simulink model "rlQuadrupedRobot"  (R2024b)
settings: Solver=ode23tb  StartTime=0.0  StopTime=10.0  RelTol=1e-3
values from neighbouring files (symbols this model uses):
  friction_force_max = mu_static * normal_force_max    [initializeRobotParameters.m]
  g = -9.81    [initializeRobotParameters.m]
  h_final = 0.75    [initializeRobotParameters.m]
  hip_eq_angle = 0    [initializeRobotParameters.m]
  init_ang_FL = d2r * quadrupedInverseKinematics(init_foot_disp_x,-init_body_height,l1,l2)    [initializeRobotParameters.m]
  init_ang_FR = init_ang_FL    [initializeRobotParameters.m]
  init_ang_RL = init_ang_FL    [initializeRobotParameters.m]
  init_ang_RR = init_ang_FL    [initializeRobotParameters.m]
  knee_eq_angle = 0    [initializeRobotParameters.m]
  l1 = 0.5517    [initializeRobotParameters.m]
  l2 = 0.5517    [initializeRobotParameters.m]
  L_back = 1.5    [initializeRobotParameters.m]
  M = 2    [initializeRobotParameters.m]
  m1 = 0.2    [initializeRobotParameters.m]
  m2 = 0.2    [initializeRobotParameters.m]
  normal_force_max = ((M+4*m1+4*m2)*abs(g))/4    [initializeRobotParameters.m]
  pitch_max = 10 * d2r    (= 0.174532925199)    [initializeRobotParameters.m]
  q_hip_max = -30 * d2r    (= -0.523598775598)    [initializeRobotParameters.m]
  q_hip_min = -120 * d2r    (= -2.09439510239)    [initializeRobotParameters.m]
  q_knee_max = 140 * d2r    (= 2.44346095279)    [initializeRobotParameters.m]
  q_knee_min = 60 * d2r    (= 1.0471975512)    [initializeRobotParameters.m]
  roll_max = 10 * d2r    (= 0.174532925199)    [initializeRobotParameters.m]
  Tf = 10    [initializeRobotParameters.m]
  Ts = 0.025    [initializeRobotParameters.m]
  u_max = 10    [initializeRobotParameters.m]
  vx_max = 2.5    [initializeRobotParameters.m]
  vy_max = 2.5    [initializeRobotParameters.m]
  vz_max = 2.5    [initializeRobotParameters.m]
  w_max = 2*pi*60/60    (= 6.28318530718)    [initializeRobotParameters.m]
  y_max = l1*cos(q_hip_max) + l2*cos(q_hip_max+q_knee_min)    [initializeRobotParameters.m]
  y_min = 0.5    [initializeRobotParameters.m]
  yaw_max = 20 * d2r    (= 0.349065850399)    [initializeRobotParameters.m]
  z_max = 0.5    [initializeRobotParameters.m]
undefined symbols (not defined in the file or in its folder): Extr_Data_LinkEndHole, Extr_Data_Mesh, ground, joint, X, Y, Z
libraries: sm_lib x113, nesl_utility x43, simulink x4, rllib x1
(part 1 of 5)
settings Model: Creator=The MathWorks, Inc.  LastModifiedBy=HP
settings SolverCC: AlgebraicLoopSolver=TrustRegion  MaxZcPerStep=1
settings OptimizationCC: ReuseModelBlockBuffer=off
settings DebuggingCC: UnconnectedInputMsg=warning  UnconnectedOutputMsg=warning  UnconnectedLineMsg=warning
settings ModelReferenceCC: EnableRefExpFcnMdlSchedulingChecks=on
settings SFSimCC: UsePrecompiledLibraries=Avoid  SimTargetLang=C++  GPUAcceleration=on  SimDLTargetLibrary=cudnn
settings RTWCC: GPUComputeCapability=3.5  DLArmComputeVersion=19.05
settings ExplorerConfigSet: InternalSimMechanicsExplorerSettings="<ExplorerConfiguration><canonicalview>default</canonicalview><AnimationSetting><BasePlaybackSpeed>1.0</BasePlaybackSpeed><PlaybackSpeedFactor>1.0</PlaybackSpeedFactor></AnimationSetting><TilePanel><TileInfo><Tiles Columns=\"1\" Count=\"1\" Rows=\"1\"><Column Weight=\"1\"/><Row Weight=\"1\"/><Tile Height=\"1\" Width=\"1\" X=\"0\" Y=\"0\"/></Tiles></TileInfo><SceneInfo><SceneViewer><BGColor><R>0.800000011920928955</R><G>0.800000011920928955</G><B>0.800000011920928955</B></BGColor><Camera><DoPerspective>off</DoPerspective><Position><X>43.366071430974273</X><Y>18.5858741674419576</Y><Z>23.6715179374704263</Z></Position><Center><X>3.63321843239613607</X><Y>-0.0564675288840452705</Y><Z>-0.89357222944397563</Z></Center><Up><X>-0.257452576685770707</X><Y>0.923486599880072756</Y><Z>-0.284412852381534909</Z></Up><ViewLimDist>1</ViewLimDist><YLim>2.82644414590933035</YLim><XLim>4.39998973134204618</XLim></Camera></SceneViewer></SceneInfo></TilePanel><MechEditorPanel><Cameras/><GfxPanelCameraMap/><VideoCreator><PlaybackSpeedRatio>1.0</PlaybackSpeedRatio><FrameRate>30</FrameRate><VideoFormat>Motion JPEG AVI</VideoFormat><FrameSize>auto</FrameSize></VideoCreator></MechEditorPanel></ExplorerConfiguration>"

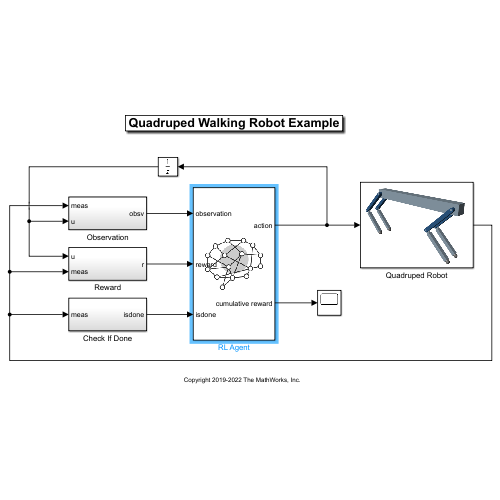
[thumbnail: Simulink's stored preview of the top-level diagram]
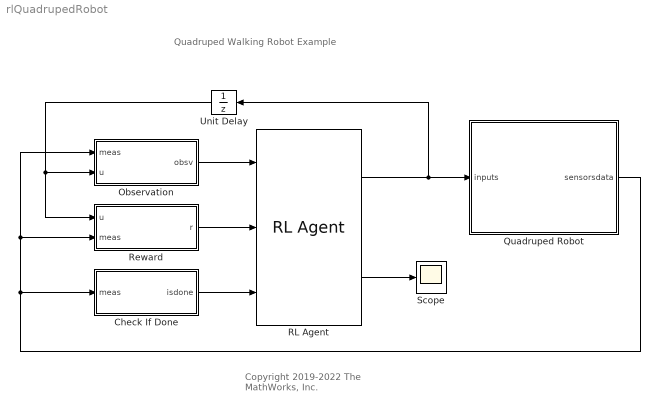
== system rlQuadrupedRobot ==
  note: Copyright 2019-2022 The MathWorks, Inc.
  note: Quadruped Walking Robot Example
  Check If Done : Subsystem
  Observation : Subsystem
  Quadruped Robot : Subsystem
      mask Display: image('$imagefile'); % Use "Edit Image" on toolstrip to change.
  RL Agent : rllib/RL Agent  Agent=agent1_Trained  ExternalActionAsInput=off  ProvideLastAction=off  ProvideCumRwd=on  TreatAsDirectFeedthrough=on  UseStrictObservationDataTypes=off
  Reward : Subsystem
  Scope : Scope
  Unit Delay : UnitDelay  SampleTime=-1  HasFrameUpgradeWarning=on
  wires:
  RL Agent/1 -> Quadruped Robot/1(inputs), Unit Delay/1
  Reward/1(r) -> RL Agent/2
  Unit Delay/1 -> Observation/2(u), Reward/1(u)
  RL Agent/2 -> Scope/1
  Quadruped Robot/1(sensorsdata) -> Observation/1(meas), Reward/2(meas), Check If Done/1(meas)
  Check If Done/1(isdone) -> RL Agent/3
  Observation/1(obsv) -> RL Agent/1

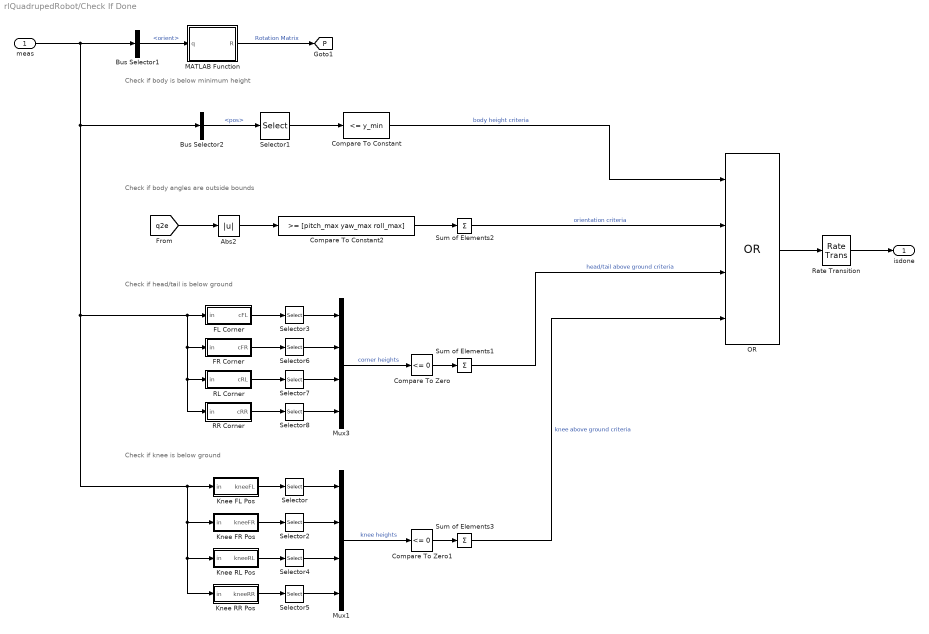
== system rlQuadrupedRobot/Check If Done ==
  note: Check if body is below minimum height
  note: Check if head/tail is below ground
  note: Check if body angles are outside bounds
  note: Check if knee is below ground
  meas : Inport
  Abs2 : Abs  ZeroCross=off  SaturateOnIntegerOverflow=off
  Bus Selector1 : BusSelector  OutputSignals=body.orient
  Bus Selector2 : BusSelector  OutputSignals=body.pos
  Compare To Constant : simulink/Logic and Bit Operations/Compare To Constant  relop=<=  const=y_min  OutDataTypeStr=boolean
  Compare To Constant2 : simulink/Logic and Bit Operations/Compare To Constant  relop=>=  const=[pitch_max yaw_max roll_max]  OutDataTypeStr=boolean
  Compare To Zero : simulink/Logic and Bit Operations/Compare To Zero  relop=<=  OutDataTypeStr=boolean
  Compare To Zero1 : simulink/Logic and Bit Operations/Compare To Zero  relop=<=  OutDataTypeStr=boolean
  FL Corner : Subsystem
  FR Corner : Subsystem
  Knee FL Pos : Subsystem
  Knee FR Pos : Subsystem
  Knee RL Pos : Subsystem
  Knee RR Pos : Subsystem
  MATLAB Function : MATLAB Function  TreatAsAtomicUnit=on
  Mux1 : Mux
  Mux3 : Mux
  OR : Logic  Operator=OR  Inputs=4  AllPortsSameDT=off  OutDataTypeStr=boolean
  RL Corner : Subsystem
  RR Corner : Subsystem
  Rate Transition : RateTransition
  Selector{,1..8} (9 alike) : Selector  InputPortWidth=3  IndexOptions=Index vector (dialog)  Indices=2  OutputSizes=1
  Sum of Elements1 : Sum  Inputs=+
  Sum of Elements2 : Sum  Inputs=+
  Sum of Elements3 : Sum  Inputs=+
  isdone : Outport  VectorParamsAs1DForOutWhenUnconnected=off
  tag scope: P=global
  wires:
  Bus Selector1/1 -> MATLAB Function/1(q)  "<orient>"
  OR/1 -> Rate Transition/1
  Rate Transition/1 -> isdone/1
  meas/1 -> Bus Selector1/1, Knee FR Pos/1(in), Knee RR Pos/1(in), Knee RL Pos/1(in), Knee FL Pos/1(in), RR Corner/1(in), RL Corner/1(in), FR Corner/1(in), FL Corner/1(in), Bus Selector2/1
  Compare To Zero1/1 -> Sum of Elements3/1
  Abs2/1 -> Compare To Constant2/1
  Compare To Constant2/1 -> Sum of Elements2/1
  Sum of Elements2/1 -> OR/2  "orientation criteria"
  Compare To Zero/1 -> Sum of Elements1/1
  MATLAB Function/1(R) -> [P]  "Rotation Matrix"
  Selector7/1 -> Mux3/3
  Mux3/1 -> Compare To Zero/1  "corner heights"
  Selector8/1 -> Mux3/4
  Selector6/1 -> Mux3/2
  RR Corner/1(cRR) -> Selector8/1
  RL Corner/1(cRL) -> Selector7/1
  Selector3/1 -> Mux3/1
  FL Corner/1(cFL) -> Selector3/1
  FR Corner/1(cFR) -> Selector6/1
  Knee FL Pos/1(kneeFL) -> Selector/1
  Selector/1 -> Mux1/1
  Selector2/1 -> Mux1/2
  Selector4/1 -> Mux1/3
  Selector5/1 -> Mux1/4
  Mux1/1 -> Compare To Zero1/1  "knee heights"
  [q2e] -> Abs2/1
  Sum of Elements1/1 -> OR/3  "head/tail above ground criteria"
  Sum of Elements3/1 -> OR/4  "knee above ground criteria"
  Knee FR Pos/1(kneeFR) -> Selector2/1
  Knee RL Pos/1(kneeRL) -> Selector4/1
  Knee RR Pos/1(kneeRR) -> Selector5/1
  Bus Selector2/1 -> Selector1/1  "<pos>"
  Compare To Constant/1 -> OR/1  "body height criteria"
  Selector1/1 -> Compare To Constant/1

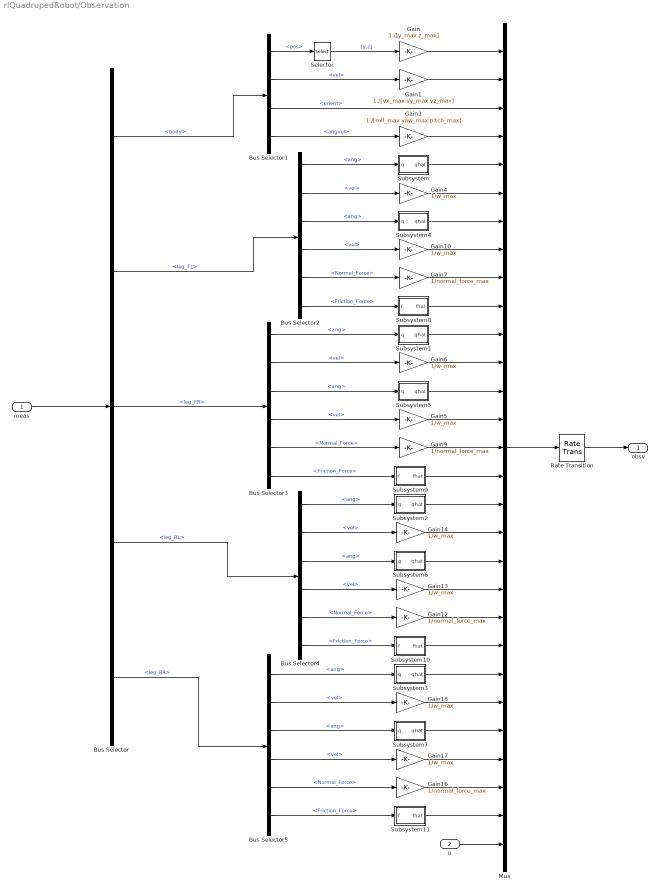
== system rlQuadrupedRobot/Observation ==
  meas : Inport
  u : Inport  Port=2
  Bus Selector : BusSelector  OutputSignals=body,leg_FL,leg_FR,leg_RL,leg_RR
  Bus Selector1 : BusSelector  OutputSignals=pos,vel,orient,angvel
  Bus Selector{2..5} (4 alike) : BusSelector  OutputSignals=hip.ang,hip.vel,knee.ang,knee.vel,foot.Normal_Force,foot.Friction_Force
  Gain : Gain  Gain=1./[y_max z_max]
  Gain1 : Gain  Gain=1./[vx_max vy_max vz_max]
  Gain{4..6,10,13..14,17..18} (8 alike) : Gain  Gain=1/w_max
  Gain{7,9,12,16} (4 alike) : Gain  Gain=1/normal_force_max
  Gain3 : Gain  Gain=1./[roll_max yaw_max pitch_max]
  Mux : Mux  Inputs=29
  Rate Transition : RateTransition
  Selector : Selector  InputPortWidth=3  IndexOptions=Index vector (dialog)  Indices=[2 3]  OutputSizes=1
  Subsystem : Subsystem
  Subsystem1 : Subsystem
  Subsystem10 : Subsystem
  Subsystem11 : Subsystem
  Subsystem2 : Subsystem
  Subsystem3 : Subsystem
  Subsystem4 : Subsystem
  Subsystem5 : Subsystem
  Subsystem6 : Subsystem
  Subsystem7 : Subsystem
  Subsystem8 : Subsystem
  Subsystem9 : Subsystem
  obsv : Outport  VectorParamsAs1DForOutWhenUnconnected=off
  wires:
  Gain3/1 -> Mux/4
  Bus Selector1/2 -> Gain1/1  "<vel>"
  Bus Selector1/1 -> Selector/1  "<pos>"
  Gain1/1 -> Mux/2
  Gain/1 -> Mux/1
  Mux/1 -> Rate Transition/1
  Bus Selector1/4 -> Gain3/1  "<angvel>"
  Selector/1 -> Gain/1  "[y,z]"
  meas/1 -> Bus Selector/1
  Bus Selector/1 -> Bus Selector1/1  "<body>"
  Bus Selector/2 -> Bus Selector2/1  "<leg_FL>"
  Bus Selector/3 -> Bus Selector3/1  "<leg_FR>"
  Bus Selector2/2 -> Gain4/1  "<vel>"
  Bus Selector/4 -> Bus Selector4/1  "<leg_RL>"
  Bus Selector/5 -> Bus Selector5/1  "<leg_RR>"
  Gain4/1 -> Mux/6
  Bus Selector2/3 -> Subsystem4/1(q)  "<ang>"
  Subsystem4/1(qhat) -> Mux/7
  Gain10/1 -> Mux/8
  Bus Selector2/4 -> Gain10/1  "<vel>"
  Bus Selector3/1 -> Subsystem1/1(q)  "<ang>"
  Bus Selector3/2 -> Gain6/1  "<vel>"
  Bus Selector3/3 -> Subsystem5/1(q)  "<ang>"
  Bus Selector3/4 -> Gain5/1  "<vel>"
  Bus Selector5/1 -> Subsystem3/1(q)  "<ang>"
  Bus Selector4/1 -> Subsystem2/1(q)  "<ang>"
  Bus Selector4/2 -> Gain14/1  "<vel>"
  Bus Selector4/3 -> Subsystem6/1(q)  "<ang>"
  Bus Selector4/4 -> Gain13/1  "<vel>"
  Bus Selector5/2 -> Gain18/1  "<vel>"
  Bus Selector5/3 -> Subsystem7/1(q)  "<ang>"
  Bus Selector5/4 -> Gain17/1  "<vel>"
  Rate Transition/1 -> obsv/1
  Bus Selector2/1 -> Subsystem/1(q)  "<ang>"
  Subsystem/1(qhat) -> Mux/5
  Bus Selector2/5 -> Gain7/1  "<Normal_Force>"
  Gain7/1 -> Mux/9
  Subsystem1/1(qhat) -> Mux/11
  Gain6/1 -> Mux/12
  Subsystem5/1(qhat) -> Mux/13
  Gain5/1 -> Mux/14
  Bus Selector3/5 -> Gain9/1  "<Normal_Force>"
  Gain9/1 -> Mux/15
  Bus Selector3/6 -> Subsystem9/1(f)  "<Friction_Force>"
  Subsystem9/1(fhat) -> Mux/16
  Gain13/1 -> Mux/20
  Subsystem6/1(qhat) -> Mux/19
  Gain14/1 -> Mux/18
  Subsystem2/1(qhat) -> Mux/17
  Bus Selector4/5 -> Gain12/1  "<Normal_Force>"
  Gain12/1 -> Mux/21
  Bus Selector4/6 -> Subsystem10/1(f)  "<Friction_Force>"
  Subsystem10/1(fhat) -> Mux/22
  Subsystem3/1(qhat) -> Mux/23
  Gain18/1 -> Mux/24
  Subsystem7/1(qhat) -> Mux/25
  Gain17/1 -> Mux/26
  Bus Selector5/5 -> Gain16/1  "<Normal_Force>"
  Gain16/1 -> Mux/27
  Bus Selector5/6 -> Subsystem11/1(f)  "<Friction_Force>"
  Subsystem11/1(fhat) -> Mux/28
  u/1 -> Mux/29
  Bus Selector2/6 -> Subsystem8/1(f)  "<Friction_Force>"
  Subsystem8/1(fhat) -> Mux/10
  Bus Selector1/3 -> Mux/3  "<orient>"

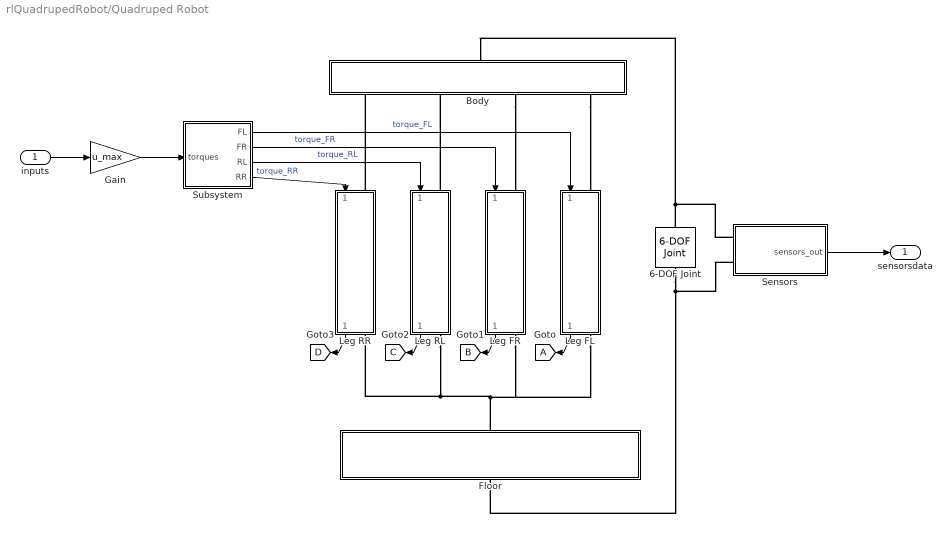
== system rlQuadrupedRobot/Quadruped Robot ==
  inputs : Inport
  6-DOF Joint : sm_lib/Joints/6-DOF Joint  JointMode=Normal  CompositeWrenchDir=FollowerOnBase  CompositeWrenchFrame=BaseFrame  SenseConstraintForce=off  SenseConstraintTorque=off  SenseTotalForce=off  SenseTotalTorque=off  PxPositionTargetSpecify=off  PxPositionTargetPriority=High  PxPositionTargetValue=0  PxPositionTargetValueUnits=m  PxVelocityTargetSpecify=on  PxVelocityTargetPriority=High  PxVelocityTargetValue=vx_init  PxVelocityTargetValueUnits=m/s  PxEquilibriumPosition=0  PxEquilibriumPositionUnits=m  PxSpringStiffness=0  PxSpringStiffnessUnits=N/m  PxDampingCoefficient=0  PxDampingCoefficientUnits=N/(m/s)  PxLowerLimitSpecify=off  PxLowerLimitBound=-1  PxLowerLimitBoundUnits=m  PxLowerLimitStiffness=1e6  PxLowerLimitStiffnessUnits=N/m  PxLowerLimitDamping=1e3  PxLowerLimitDampingUnits=N/(m/s)  PxLowerLimitTransitionRegionWidth=1e-4  PxLowerLimitTransitionRegionWidthUnits=m  PxUpperLimitSpecify=off  PxUpperLimitBound=1  PxUpperLimitBoundUnits=m  PxUpperLimitStiffness=1e6  PxUpperLimitStiffnessUnits=N/m  PxUpperLimitDamping=1e3  PxUpperLimitDampingUnits=N/(m/s)  PxUpperLimitTransitionRegionWidth=1e-4  PxUpperLimitTransitionRegionWidthUnits=m  PxTorqueActuationMode=NoTorque  PxMotionActuationMode=ComputedMotion  PxSensePosition=off  PxSenseVelocity=off  PxSenseAcceleration=off  PxSenseTorqueForce=off  PxSenseLowerLimitTorqueForce=off  PxSenseUpperLimitTorqueForce=off  PyPositionTargetSpecify=on  PyPositionTargetPriority=High  PyPositionTargetValue=y_init  PyPositionTargetValueUnits=m  PyVelocityTargetSpecify=on  PyVelocityTargetPriority=High  PyVelocityTargetValue=vy_init  PyVelocityTargetValueUnits=m/s  PyEquilibriumPosition=0  PyEquilibriumPositionUnits=m  PySpringStiffness=0  PySpringStiffnessUnits=N/m  PyDampingCoefficient=0  PyDampingCoefficientUnits=N/(m/s)  PyLowerLimitSpecify=off  PyLowerLimitBound=-1  PyLowerLimitBoundUnits=m  PyLowerLimitStiffness=1e6  PyLowerLimitStiffnessUnits=N/m  PyLowerLimitDamping=1e3  PyLowerLimitDampingUnits=N/(m/s)  PyLowerLimitTransitionRegionWidth=1e-4  PyLowerLimitTransitionRegionWidthUnits=m  PyUpperLimitSpecify=off  PyUpperLimitBound=1  PyUpperLimitBoundUnits=m  PyUpperLimitStiffness=1e6  PyUpperLimitStiffnessUnits=N/m  PyUpperLimitDamping=1e3  PyUpperLimitDampingUnits=N/(m/s)  PyUpperLimitTransitionRegionWidth=1e-4  PyUpperLimitTransitionRegionWidthUnits=m  PyTorqueActuationMode=NoTorque  PyMotionActuationMode=ComputedMotion  PySensePosition=off  PySenseVelocity=off  PySenseAcceleration=off  PySenseTorqueForce=off  PySenseLowerLimitTorqueForce=off  PySenseUpperLimitTorqueForce=off  PzPositionTargetSpecify=off  PzPositionTargetPriority=High  PzPositionTargetValue=0  PzPositionTargetValueUnits=m  PzVelocityTargetSpecify=on  PzVelocityTargetPriority=High  PzVelocityTargetValue=0  PzVelocityTargetValueUnits=m/s  PzEquilibriumPosition=0  PzEquilibriumPositionUnits=m  PzSpringStiffness=0  PzSpringStiffnessUnits=N/m  PzDampingCoefficient=0  PzDampingCoefficientUnits=N/(m/s)  PzLowerLimitSpecify=off  PzLowerLimitBound=-1  PzLowerLimitBoundUnits=m  PzLowerLimitStiffness=1e6  PzLowerLimitStiffnessUnits=N/m  PzLowerLimitDamping=1e3  PzLowerLimitDampingUnits=N/(m/s)  PzLowerLimitTransitionRegionWidth=1e-4  PzLowerLimitTransitionRegionWidthUnits=m  PzUpperLimitSpecify=off  PzUpperLimitBound=1  PzUpperLimitBoundUnits=m  PzUpperLimitStiffness=1e6  PzUpperLimitStiffnessUnits=N/m  PzUpperLimitDamping=1e3  PzUpperLimitDampingUnits=N/(m/s)  PzUpperLimitTransitionRegionWidth=1e-4  PzUpperLimitTransitionRegionWidthUnits=m  PzTorqueActuationMode=NoTorque  PzMotionActuationMode=ComputedMotion  PzSensePosition=off  PzSenseVelocity=off  PzSenseAcceleration=off  PzSenseTorqueForce=off  PzSenseLowerLimitTorqueForce=off  PzSenseUpperLimitTorqueForce=off  SphPositionTargetSpecify=off  SphPositionTargetPriority=High  SphPositionTargetRotationMethod=None  SphPositionTargetFollAlignAxisA=+X  SphPositionTargetBaseAlignAxisA=+Y  SphPositionTargetFollAlignAxisB=+Y  SphPositionTargetBaseAlignAxisB=+Z  SphPositionTargetRotationStandardAxis=+Z  SphPositionTargetRotationAngle=0.0  SphPositionTargetRotationAngleUnits=deg  SphPositionTargetRotationArbitraryAxis=[0 0 1]  SphPositionTargetRotationSequenceAxes=FollowerAxes  SphPositionTargetRotationSequence=XYX  SphPositionTargetRotationSequenceAngles=[0 0 0]  SphPositionTargetRotationSequenceAnglesUnits=deg  SphPositionTargetRotationMatrix=[1 0 0; 0 1 0; 0 0 1]  SphPositionTargetQuaternion=[1 0 0 0]  SphVelocityTargetSpecify=off  SphVelocityTargetPriority=High  SphVelocityTargetValue=[0 0 0]  SphVelocityTargetValueUnits=deg/s  SphVelocityTargetInFollowerFrame=on  SphEqPosRotationMethod=None  SphEqPosFollAlignAxisA=+X  SphEqPosBaseAlignAxisA=+Y  SphEqPosFollAlignAxisB=+Y  SphEqPosBaseAlignAxisB=+Z  SphEqPosRotationStandardAxis=+Z  SphEqPosRotationAngle=0.0  SphEqPosRotationAngleUnits=deg  SphEqPosRotationArbitraryAxis=[0 0 1]  SphEqPosRotationSequenceAxes=FollowerAxes  SphEqPosRotationSequence=XYX  SphEqPosRotationSequenceAngles=[0 0 0]  SphEqPosRotationSequenceAnglesUnits=deg  SphEqPosRotationMatrix=[1 0 0; 0 1 0; 0 0 1]  SphEqPosQuaternion=[1 0 0 0]  SphSpringStiffness=0  SphSpringStiffnessUnits=N*m/deg  SphDampingCoefficient=0  SphDampingCoefficientUnits=N*m/(deg/s)  SphLowerLimitSpecify=off  SphLowerLimitBound=15  SphLowerLimitBoundUnits=deg  SphLowerLimitStiffness=1e4  SphLowerLimitStiffnessUnits=N*m/deg  SphLowerLimitDamping=10  SphLowerLimitDampingUnits=N*m/(deg/s)  SphLowerLimitTransitionRegionWidth=0.1  SphLowerLimitTransitionRegionWidthUnits=deg  SphUpperLimitSpecify=off  SphUpperLimitBound=45  SphUpperLimitBoundUnits=deg  SphUpperLimitStiffness=1e4  SphUpperLimitStiffnessUnits=N*m/deg  SphUpperLimitDamping=10  SphUpperLimitDampingUnits=N*m/(deg/s)  SphUpperLimitTransitionRegionWidth=0.1  SphUpperLimitTransitionRegionWidthUnits=deg  SphTorqueActuationMode=NoTorque  SphActuateTorqueX=off  SphActuateTorqueY=off  SphActuateTorqueZ=off  SphActuateTorque=off  SphActuationFrame=BaseFrame  SphSensePosition=off  SphSenseVelocityX=off  SphSenseVelocityY=off  SphSenseVelocityZ=off  SphSenseVelocity=off  SphSenseAccelerationX=off  SphSenseAccelerationY=off  SphSenseAccelerationZ=off  SphSenseAcceleration=off  SphSenseLowerLimitTorqueMag=off  SphSenseUpperLimitTorqueMag=off  SphSensingFrame=BaseFrame
  Body : Subsystem  Tag=CustomStyle
      mask Display: image('$imagefile'); % Use "Edit Image" on toolstrip to change.
  Floor : Subsystem
  Gain : Gain  Gain=u_max
  Goto : Goto  TagVisibility=global
  Leg FL : Subsystem  Tag=PublishSubsystemCustomStyle  mask{leg_type=Front Left, leg_width=0.1*l1, th1_0=init_ang_FL(1), th1_dot_0=0, eqAngle_hip=hip_eq_angle, k_hip=joint.stiffness, b_hip=joint.damping, klim_hip=joint.limitStiffness, blim_hip=joint.limitDamping, tr_width_hip=joint.transitionWidth, th2_0=init_ang_FL(2), th2_dot_0=0, eqAngle_knee=knee_eq_angle, k_knee=joint.stiffness, b_knee=joint.damping, klim_knee=joint.limitStiffness, blim_knee=joint.limitDamping, tr_width_knee=joint.transitionWidth}
      mask prompts: leg_type "Leg type"; leg_width "Leg width (m)"; th1_0 "Initial hip angle (rad)"; th1_dot_0 "Initial hip angular velocity (rad/s)"; eqAngle_hip "Equilibrium Angle (rad)"; k_hip "Joint Stiffness (N/m)"; b_hip "Joint Damping (Ns/m)"; klim_hip "Joint Limit Stiffness (N/m)"; blim_hip "Joint Limit Damping (Ns/m)"; tr_width_hip "Transition Width (rad)"; th2_0 "Initial knee angle (rad)"; th2_dot_0 "Initial knee angular velocity (rad/s)"; eqAngle_knee "Equilibrium Angle (rad)"; k_knee "Joint Stiffness (N/m)"; b_knee "Joint Damping (Ns/m)"; klim_knee "Joint Limit Stiffness (N/m)"; blim_knee "Joint Limit Damping (Ns/m)"; tr_width_knee "Transition Width (rad)"
      mask init:
      | if (leg_type == 1 || leg_type == 3)
      |     sideSign = -1;
      | else
      |     sideSign = 1;
      | end
      mask TypeOptions leg_type: Front Left | Front Right | Rear Left | Rear Right
      mask DialogControl Container4 Prompt: Hip Joint
      mask DialogControl Container7 Prompt: Knee Joint
      mask Display: image('$imagefile'); % Use "Edit Image" on toolstrip to change.
  Leg FR : Subsystem  Tag=CustomStyle  mask{leg_type=Front Right, leg_width=0.1*l1, th1_0=init_ang_FR(1), th1_dot_0=0, eqAngle_hip=hip_eq_angle, k_hip=joint.stiffness, b_hip=joint.damping, klim_hip=joint.limitStiffness, blim_hip=joint.limitDamping, tr_width_hip=joint.transitionWidth, th2_0=init_ang_FR(2), th2_dot_0=0, eqAngle_knee=knee_eq_angle, k_knee=joint.stiffness, b_knee=joint.damping, klim_knee=joint.limitStiffness, blim_knee=joint.limitDamping, tr_width_knee=joint.transitionWidth}
      mask prompts: leg_type "Leg type"; leg_width "Leg width (m)"; th1_0 "Initial hip angle (rad)"; th1_dot_0 "Initial hip angular velocity (rad/s)"; eqAngle_hip "Equilibrium Angle (rad)"; k_hip "Joint Stiffness (N/m)"; b_hip "Joint Damping (Ns/m)"; klim_hip "Joint Limit Stiffness (N/m)"; blim_hip "Joint Limit Damping (Ns/m)"; tr_width_hip "Transition Width (rad)"; th2_0 "Initial knee angle (rad)"; th2_dot_0 "Initial knee angular velocity (rad/s)"; eqAngle_knee "Equilibrium Angle (rad)"; k_knee "Joint Stiffness (N/m)"; b_knee "Joint Damping (Ns/m)"; klim_knee "Joint Limit Stiffness (N/m)"; blim_knee "Joint Limit Damping (Ns/m)"; tr_width_knee "Transition Width (rad)"
      mask init:
      | if (leg_type == 1 || leg_type == 3)
      |     sideSign = -1;
      | else
      |     sideSign = 1;
      | end
      mask TypeOptions leg_type: Front Left | Front Right | Rear Left | Rear Right
      mask DialogControl Container4 Prompt: Hip Joint
      mask DialogControl Container7 Prompt: Knee Joint
      mask Display: image('$imagefile'); % Use "Edit Image" on toolstrip to change.
  Leg RL : Subsystem  Tag=CustomStyle  mask{leg_type=Rear Left, leg_width=0.1*l1, th1_0=init_ang_RL(1), th1_dot_0=0, eqAngle_hip=hip_eq_angle, k_hip=joint.stiffness, b_hip=joint.damping, klim_hip=joint.limitStiffness, blim_hip=joint.limitDamping, tr_width_hip=joint.transitionWidth, th2_0=init_ang_RL(2), th2_dot_0=0, eqAngle_knee=knee_eq_angle, k_knee=joint.stiffness, b_knee=joint.damping, klim_knee=joint.limitStiffness, blim_knee=joint.limitDamping, tr_width_knee=joint.transitionWidth}
      mask prompts: leg_type "Leg type"; leg_width "Leg width (m)"; th1_0 "Initial hip angle (rad)"; th1_dot_0 "Initial hip angular velocity (rad/s)"; eqAngle_hip "Equilibrium Angle (rad)"; k_hip "Joint Stiffness (N/m)"; b_hip "Joint Damping (Ns/m)"; klim_hip "Joint Limit Stiffness (N/m)"; blim_hip "Joint Limit Damping (Ns/m)"; tr_width_hip "Transition Width (rad)"; th2_0 "Initial knee angle (rad)"; th2_dot_0 "Initial knee angular velocity (rad/s)"; eqAngle_knee "Equilibrium Angle (rad)"; k_knee "Joint Stiffness (N/m)"; b_knee "Joint Damping (Ns/m)"; klim_knee "Joint Limit Stiffness (N/m)"; blim_knee "Joint Limit Damping (Ns/m)"; tr_width_knee "Transition Width (rad)"
      mask init:
      | if (leg_type == 1 || leg_type == 3)
      |     sideSign = -1;
      | else
      |     sideSign = 1;
      | end
      mask TypeOptions leg_type: Front Left | Front Right | Rear Left | Rear Right
      mask DialogControl Container4 Prompt: Hip Joint
      mask DialogControl Container7 Prompt: Knee Joint
      mask Display: image('$imagefile'); % Use "Edit Image" on toolstrip to change.
  Leg RR : Subsystem  Tag=CustomStyle  mask{leg_type=Rear Right, leg_width=0.1*l1, th1_0=init_ang_RR(1), th1_dot_0=0, eqAngle_hip=hip_eq_angle, k_hip=joint.stiffness, b_hip=joint.damping, klim_hip=joint.limitStiffness, blim_hip=joint.limitDamping, tr_width_hip=joint.transitionWidth, th2_0=init_ang_RR(2), th2_dot_0=0, eqAngle_knee=knee_eq_angle, k_knee=joint.stiffness, b_knee=joint.damping, klim_knee=joint.limitStiffness, blim_knee=joint.limitDamping, tr_width_knee=joint.transitionWidth}
      mask prompts: leg_type "Leg type"; leg_width "Leg width (m)"; th1_0 "Initial hip angle (rad)"; th1_dot_0 "Initial hip angular velocity (rad/s)"; eqAngle_hip "Equilibrium Angle (rad)"; k_hip "Joint Stiffness (N/m)"; b_hip "Joint Damping (Ns/m)"; klim_hip "Joint Limit Stiffness (N/m)"; blim_hip "Joint Limit Damping (Ns/m)"; tr_width_hip "Transition Width (rad)"; th2_0 "Initial knee angle (rad)"; th2_dot_0 "Initial knee angular velocity (rad/s)"; eqAngle_knee "Equilibrium Angle (rad)"; k_knee "Joint Stiffness (N/m)"; b_knee "Joint Damping (Ns/m)"; klim_knee "Joint Limit Stiffness (N/m)"; blim_knee "Joint Limit Damping (Ns/m)"; tr_width_knee "Transition Width (rad)"
      mask init:
      | if (leg_type == 1 || leg_type == 3)
      |     sideSign = -1;
      | else
      |     sideSign = 1;
      | end
      mask TypeOptions leg_type: Front Left | Front Right | Rear Left | Rear Right
      mask DialogControl Container4 Prompt: Hip Joint
      mask DialogControl Container7 Prompt: Knee Joint
      mask Display: image('$imagefile'); % Use "Edit Image" on toolstrip to change.
  Sensors : Subsystem
  Subsystem : Subsystem
  sensorsdata : Outport  VectorParamsAs1DForOutWhenUnconnected=off
  tag scope: B=global, C=global, D=global
  wires:
  inputs/1 -> Gain/1
  Subsystem/1(FL) -> Leg FL/1(torque)  "torque_FL"
  Subsystem/2(FR) -> Leg FR/1(torque)  "torque_FR"
  Subsystem/3(RL) -> Leg RL/1(torque)  "torque_RL"
  Subsystem/4(RR) -> Leg RR/1(torque)  "torque_RR"
  Leg FL/1(sensors) -> Goto/1
  Leg FR/1(sensors) -> [B]
  Leg RL/1(sensors) -> [C]
  Leg RR/1(sensors) -> [D]
  Sensors/1(sensors_out) -> sensorsdata/1
  Gain/1 -> Subsystem/1(torques)
  connections:
  6-DOF Joint/RConn1 -- Body/RConn1 -- Sensors/LConn1
  Leg RR/LConn1 -- Body/LConn1
  Leg RL/LConn1 -- Body/LConn2
  Body/LConn3 -- Leg FR/LConn1
  Body/LConn4 -- Leg FL/LConn1
  Sensors/LConn2 -- Floor/LConn1 -- 6-DOF Joint/LConn1
  Floor/RConn1 -- Leg FL/RConn1 -- Leg FR/RConn1 -- Leg RL/RConn1 -- Leg RR/RConn1

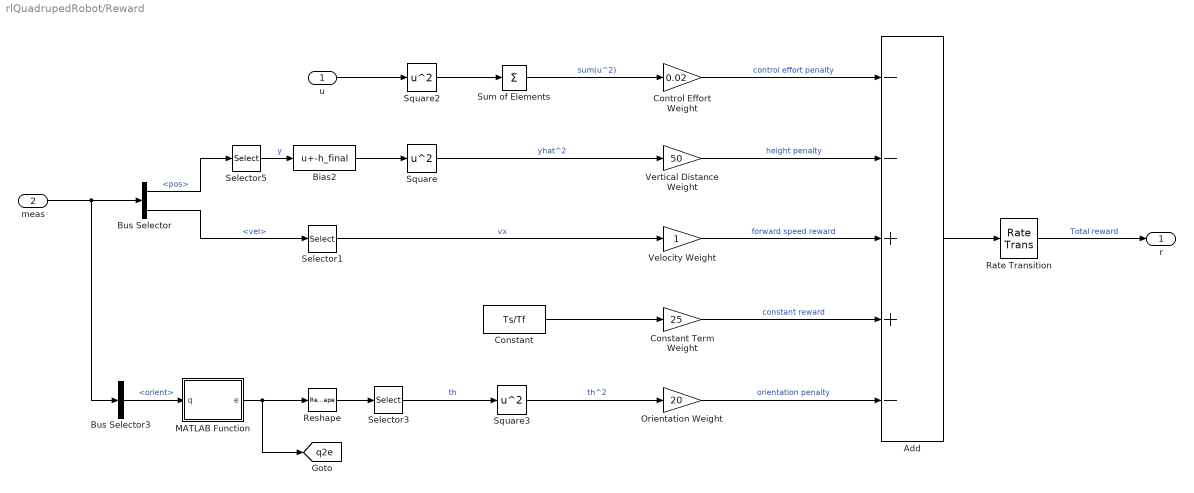
== system rlQuadrupedRobot/Reward ==
  u : Inport
  meas : Inport  Port=2
  Add : Sum  Inputs=--++-
  Bias2 : Bias  Bias=-h_final  SaturateOnIntegerOverflow=off
  Bus Selector : BusSelector  OutputSignals=body.pos,body.vel
  Bus Selector3 : BusSelector  OutputSignals=body.orient
  "Constant " : Constant  Value=Ts/Tf  SampleTime=-1
  Constant Term Weight : Gain  Gain=25
  Control Effort Weight : Gain  Gain=0.02
  MATLAB Function : MATLAB Function  TreatAsAtomicUnit=on
  Orientation Weight : Gain  Gain=20
  Rate Transition : RateTransition
  Reshape : Reshape
  Selector1 : Selector  InputPortWidth=3  IndexOptions=Index vector (dialog)  Indices=1  OutputSizes=1
  Selector3 : Selector  InputPortWidth=3  IndexOptions=Index vector (dialog)  Indices=1  OutputSizes=1
  Selector5 : Selector  InputPortWidth=3  IndexOptions=Index vector (dialog)  Indices=2  OutputSizes=1
  Square : Math  Operator=square
  Square2 : Math  Operator=square  SignedPower=on
  Square3 : Math  Operator=square  SignedPower=on
  Sum of Elements : Sum  Inputs=+  OutDataTypeStr=double
  Velocity Weight : Gain
  Vertical Distance Weight : Gain  Gain=50
  r : Outport  VectorParamsAs1DForOutWhenUnconnected=off
  tag scope: q2e=global
  wires:
  Selector5/1 -> Bias2/1  "y"
  Square/1 -> Vertical Distance Weight/1  "yhat^2"
  Bus Selector/2 -> Selector1/1  "<vel>"
  Sum of Elements/1 -> Control Effort Weight/1  "sum(u^2)"
  Add/1 -> Rate Transition/1
  Bus Selector/1 -> Selector5/1  "<pos>"
  meas/1 -> Bus Selector3/1, Bus Selector/1
  Velocity Weight/1 -> Add/3  "forward speed reward"
  Control Effort Weight/1 -> Add/1  "control effort penalty"
  Selector1/1 -> Velocity Weight/1  "vx"
  "Constant "/1 -> Constant Term Weight/1
  Square2/1 -> Sum of Elements/1
  Vertical Distance Weight/1 -> Add/2  "height penalty"
  Rate Transition/1 -> r/1  "Total reward"
  Bus Selector3/1 -> MATLAB Function/1(q)  "<orient>"
  Reshape/1 -> Selector3/1
  Constant Term Weight/1 -> Add/4  "constant reward"
  Orientation Weight/1 -> Add/5  "orientation penalty"
  Square3/1 -> Orientation Weight/1  "th^2"
  Selector3/1 -> Square3/1  "th"
  Bias2/1 -> Square/1
  MATLAB Function/1(e) -> [q2e], Reshape/1
  u/1 -> Square2/1

== system rlQuadrupedRobot/Check If Done/FL Corner ==
  in : Inport
  Add : Sum
  Bus Selector1 : BusSelector  OutputSignals=body.pos
  Constant1 : Constant  Value=L_back*[0.5; -0.5*0.1; 0.5*0.1]  SampleTime=-1
  Product : Product  Multiplication=Matrix(*)
  cFL : Outport  VectorParamsAs1DForOutWhenUnconnected=off
  wires:
  in/1 -> Bus Selector1/1
  Bus Selector1/1 -> Add/1  "<pos>"
  Add/1 -> cFL/1
  [P] -> Product/1
  Product/1 -> Add/2  "corner pos w.r.t. cg"
  Constant1/1 -> Product/2

== system rlQuadrupedRobot/Check If Done/FR Corner ==
  in : Inport
  Add : Sum
  Bus Selector1 : BusSelector  OutputSignals=body.pos
  Constant1 : Constant  Value=L_back*[0.5; -0.5*0.1; -0.5*0.1]  SampleTime=-1
  Product : Product  Multiplication=Matrix(*)
  cFR : Outport  VectorParamsAs1DForOutWhenUnconnected=off
  wires:
  Bus Selector1/1 -> Add/1  "<pos>"
  in/1 -> Bus Selector1/1
  Product/1 -> Add/2  "corner pos w.r.t. cg"
  Add/1 -> cFR/1
  Constant1/1 -> Product/2
  [P] -> Product/1

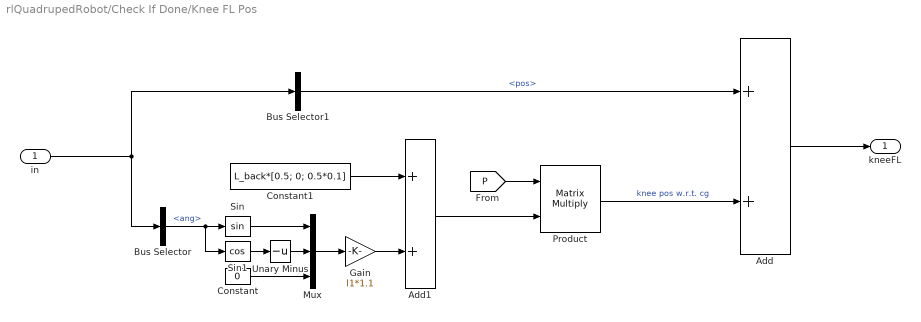
== system rlQuadrupedRobot/Check If Done/Knee FL Pos ==
  in : Inport
  Add : Sum
  Add1 : Sum
  Bus Selector : BusSelector  OutputSignals=leg_FL.hip.ang
  Bus Selector1 : BusSelector  OutputSignals=body.pos
  Constant : Constant  Value=0  SampleTime=-1
  Constant1 : Constant  Value=L_back*[0.5; 0; 0.5*0.1]  SampleTime=-1
  Gain : Gain  Gain=l1*1.1
  Mux : Mux  Inputs=3
  Product : Product  Multiplication=Matrix(*)
  Sin : Trigonometry
  Sin1 : Trigonometry  Operator=cos
  Unary Minus : UnaryMinus
  kneeFL : Outport  VectorParamsAs1DForOutWhenUnconnected=off
  wires:
  Sin/1 -> Mux/1
  Sin1/1 -> Unary Minus/1
  Mux/1 -> Gain/1
  Constant/1 -> Mux/3
  in/1 -> Bus Selector/1, Bus Selector1/1
  Bus Selector/1 -> Sin1/1, Sin/1  "<ang>"
  Bus Selector1/1 -> Add/1  "<pos>"
  Add/1 -> kneeFL/1
  Gain/1 -> Add1/2
  [P] -> Product/1
  Product/1 -> Add/2  "knee pos w.r.t. cg"
  Constant1/1 -> Add1/1
  Add1/1 -> Product/2
  Unary Minus/1 -> Mux/2

== system rlQuadrupedRobot/Check If Done/Knee FR Pos ==
  in : Inport
  Add : Sum
  Add1 : Sum
  Bus Selector : BusSelector  OutputSignals=leg_FR.hip.ang
  Bus Selector1 : BusSelector  OutputSignals=body.pos
  Constant : Constant  Value=0  SampleTime=-1
  Constant1 : Constant  Value=L_back*[0.5; 0; -0.5*0.1]  SampleTime=-1
  Gain : Gain  Gain=l1*1.1
  Mux : Mux  Inputs=3
  Product : Product  Multiplication=Matrix(*)
  Sin : Trigonometry
  Sin1 : Trigonometry  Operator=cos
  Unary Minus : UnaryMinus
  kneeFR : Outport  VectorParamsAs1DForOutWhenUnconnected=off
  wires:
  Add1/1 -> Product/2
  Bus Selector1/1 -> Add/1  "<pos>"
  in/1 -> Bus Selector/1, Bus Selector1/1
  Bus Selector/1 -> Sin1/1, Sin/1  "<ang>"
  Product/1 -> Add/2  "knee pos w.r.t. cg"
  Add/1 -> kneeFR/1
  Gain/1 -> Add1/2
  Sin1/1 -> Unary Minus/1
  Constant/1 -> Mux/3
  Constant1/1 -> Add1/1
  Mux/1 -> Gain/1
  Sin/1 -> Mux/1
  Unary Minus/1 -> Mux/2
  [P] -> Product/1

== system rlQuadrupedRobot/Check If Done/Knee RL Pos ==
  in : Inport
  Add : Sum
  Add1 : Sum
  Bus Selector : BusSelector  OutputSignals=leg_RL.hip.ang
  Bus Selector1 : BusSelector  OutputSignals=body.pos
  Constant : Constant  Value=0  SampleTime=-1
  Constant1 : Constant  Value=L_back*[-0.5; 0; 0.5*0.1]  SampleTime=-1
  Gain : Gain  Gain=l1*1.1
  Mux : Mux  Inputs=3
  Product : Product  Multiplication=Matrix(*)
  Sin : Trigonometry
  Sin1 : Trigonometry  Operator=cos
  Unary Minus : UnaryMinus
  kneeRL : Outport  VectorParamsAs1DForOutWhenUnconnected=off
  wires:
  Add1/1 -> Product/2
  Bus Selector1/1 -> Add/1  "<pos>"
  in/1 -> Bus Selector/1, Bus Selector1/1
  Bus Selector/1 -> Sin1/1, Sin/1  "<ang>"
  Product/1 -> Add/2  "knee pos w.r.t. cg"
  Add/1 -> kneeRL/1
  Gain/1 -> Add1/2
  Sin1/1 -> Unary Minus/1
  Constant/1 -> Mux/3
  Constant1/1 -> Add1/1
  Mux/1 -> Gain/1
  Sin/1 -> Mux/1
  Unary Minus/1 -> Mux/2
  [P] -> Product/1

== system rlQuadrupedRobot/Check If Done/Knee RR Pos ==
  in : Inport
  Add : Sum
  Add1 : Sum
  Bus Selector : BusSelector  OutputSignals=leg_RR.hip.ang
  Bus Selector1 : BusSelector  OutputSignals=body.pos
  Constant : Constant  Value=0  SampleTime=-1
  Constant1 : Constant  Value=L_back*[-0.5; 0; -0.5*0.1]  SampleTime=-1
  Gain : Gain  Gain=l1*1.1
  Mux : Mux  Inputs=3
  Product : Product  Multiplication=Matrix(*)
  Sin : Trigonometry
  Sin1 : Trigonometry  Operator=cos
  Unary Minus : UnaryMinus
  kneeRR : Outport  VectorParamsAs1DForOutWhenUnconnected=off
  wires:
  Add1/1 -> Product/2
  Bus Selector1/1 -> Add/1  "<pos>"
  in/1 -> Bus Selector/1, Bus Selector1/1
  Bus Selector/1 -> Sin1/1, Sin/1  "<ang>"
  Product/1 -> Add/2  "knee pos w.r.t. cg"
  Add/1 -> kneeRR/1
  Gain/1 -> Add1/2
  Sin1/1 -> Unary Minus/1
  Constant/1 -> Mux/3
  Constant1/1 -> Add1/1
  Mux/1 -> Gain/1
  Sin/1 -> Mux/1
  Unary Minus/1 -> Mux/2
  [P] -> Product/1

== system rlQuadrupedRobot/Check If Done/RL Corner ==
  in : Inport
  Add : Sum
  Bus Selector1 : BusSelector  OutputSignals=body.pos
  Constant1 : Constant  Value=L_back*[-0.5; 0.5*0.1; 0.5*0.1]  SampleTime=-1
  Product : Product  Multiplication=Matrix(*)
  cRL : Outport  VectorParamsAs1DForOutWhenUnconnected=off
  wires:
  Constant1/1 -> Product/2
  Bus Selector1/1 -> Add/1  "<pos>"
  in/1 -> Bus Selector1/1
  Product/1 -> Add/2  "corner pos w.r.t. cg"
  Add/1 -> cRL/1
  [P] -> Product/1

== system rlQuadrupedRobot/Check If Done/RR Corner ==
  in : Inport
  Add : Sum
  Bus Selector1 : BusSelector  OutputSignals=body.pos
  Constant1 : Constant  Value=L_back*[-0.5; -0.5*0.1; -0.5*0.1]  SampleTime=-1
  Product : Product  Multiplication=Matrix(*)
  cRR : Outport  VectorParamsAs1DForOutWhenUnconnected=off
  wires:
  Constant1/1 -> Product/2
  Bus Selector1/1 -> Add/1  "<pos>"
  in/1 -> Bus Selector1/1
  Product/1 -> Add/2  "corner pos w.r.t. cg"
  Add/1 -> cRR/1
  [P] -> Product/1

== system rlQuadrupedRobot/Observation/Subsystem ==
  q : Inport
  Bias : Bias  Bias=-q_hip_min  SaturateOnIntegerOverflow=off
  Bias1 : Bias  Bias=-1  SaturateOnIntegerOverflow=off
  Gain8 : Gain  Gain=2/(q_hip_max-q_hip_min)
  qhat : Outport  VectorParamsAs1DForOutWhenUnconnected=off
  wires:
  q/1 -> Bias/1
  Bias/1 -> Gain8/1
  Gain8/1 -> Bias1/1
  Bias1/1 -> qhat/1

== system rlQuadrupedRobot/Observation/Subsystem1 ==
  q : Inport
  Bias : Bias  Bias=-q_hip_min  SaturateOnIntegerOverflow=off
  Bias1 : Bias  Bias=-1  SaturateOnIntegerOverflow=off
  Gain8 : Gain  Gain=2/(q_hip_max-q_hip_min)
  qhat : Outport  VectorParamsAs1DForOutWhenUnconnected=off
  wires:
  Bias1/1 -> qhat/1
  Gain8/1 -> Bias1/1
  Bias/1 -> Gain8/1
  q/1 -> Bias/1

== system rlQuadrupedRobot/Observation/Subsystem10 ==
  f : Inport
  Gain8 : Gain  Gain=1/friction_force_max
  Sqrt : Sqrt
  Square : Math  Operator=square  SignedPower=on
  Sum of Elements : Sum  Inputs=+
  fhat : Outport  VectorParamsAs1DForOutWhenUnconnected=off
  wires:
  f/1 -> Gain8/1
  Gain8/1 -> Square/1
  Square/1 -> Sum of Elements/1
  Sum of Elements/1 -> Sqrt/1
  Sqrt/1 -> fhat/1

== system rlQuadrupedRobot/Observation/Subsystem11 ==
  f : Inport
  Gain8 : Gain  Gain=1/friction_force_max
  Sqrt : Sqrt
  Square : Math  Operator=square  SignedPower=on
  Sum of Elements : Sum  Inputs=+
  fhat : Outport  VectorParamsAs1DForOutWhenUnconnected=off
  wires:
  f/1 -> Gain8/1
  Gain8/1 -> Square/1
  Square/1 -> Sum of Elements/1
  Sum of Elements/1 -> Sqrt/1
  Sqrt/1 -> fhat/1

== system rlQuadrupedRobot/Observation/Subsystem2 ==
  q : Inport
  Bias : Bias  Bias=-q_hip_min  SaturateOnIntegerOverflow=off
  Bias1 : Bias  Bias=-1  SaturateOnIntegerOverflow=off
  Gain8 : Gain  Gain=2/(q_hip_max-q_hip_min)
  qhat : Outport  VectorParamsAs1DForOutWhenUnconnected=off
  wires:
  Bias1/1 -> qhat/1
  Gain8/1 -> Bias1/1
  Bias/1 -> Gain8/1
  q/1 -> Bias/1

== system rlQuadrupedRobot/Observation/Subsystem3 ==
  q : Inport
  Bias : Bias  Bias=-q_hip_min  SaturateOnIntegerOverflow=off
  Bias1 : Bias  Bias=-1  SaturateOnIntegerOverflow=off
  Gain8 : Gain  Gain=2/(q_hip_max-q_hip_min)
  qhat : Outport  VectorParamsAs1DForOutWhenUnconnected=off
  wires:
  Bias1/1 -> qhat/1
  Gain8/1 -> Bias1/1
  Bias/1 -> Gain8/1
  q/1 -> Bias/1

== system rlQuadrupedRobot/Observation/Subsystem4 ==
  q : Inport
  Bias : Bias  Bias=-q_knee_min  SaturateOnIntegerOverflow=off
  Bias1 : Bias  Bias=-1  SaturateOnIntegerOverflow=off
  Gain8 : Gain  Gain=2/(q_knee_max-q_knee_min)
  qhat : Outport  VectorParamsAs1DForOutWhenUnconnected=off
  wires:
  Bias1/1 -> qhat/1
  Gain8/1 -> Bias1/1
  Bias/1 -> Gain8/1
  q/1 -> Bias/1

== system rlQuadrupedRobot/Observation/Subsystem5 ==
  q : Inport
  Bias : Bias  Bias=-q_knee_min  SaturateOnIntegerOverflow=off
  Bias1 : Bias  Bias=-1  SaturateOnIntegerOverflow=off
  Gain8 : Gain  Gain=2/(q_knee_max-q_knee_min)
  qhat : Outport  VectorParamsAs1DForOutWhenUnconnected=off
  wires:
  Bias1/1 -> qhat/1
  Gain8/1 -> Bias1/1
  Bias/1 -> Gain8/1
  q/1 -> Bias/1

== system rlQuadrupedRobot/Observation/Subsystem6 ==
  q : Inport
  Bias : Bias  Bias=-q_knee_min  SaturateOnIntegerOverflow=off
  Bias1 : Bias  Bias=-1  SaturateOnIntegerOverflow=off
  Gain8 : Gain  Gain=2/(q_knee_max-q_knee_min)
  qhat : Outport  VectorParamsAs1DForOutWhenUnconnected=off
  wires:
  Bias1/1 -> qhat/1
  Gain8/1 -> Bias1/1
  Bias/1 -> Gain8/1
  q/1 -> Bias/1

== system rlQuadrupedRobot/Observation/Subsystem7 ==
  q : Inport
  Bias : Bias  Bias=-q_knee_min  SaturateOnIntegerOverflow=off
  Bias1 : Bias  Bias=-1  SaturateOnIntegerOverflow=off
  Gain8 : Gain  Gain=2/(q_knee_max-q_knee_min)
  qhat : Outport  VectorParamsAs1DForOutWhenUnconnected=off
  wires:
  Bias1/1 -> qhat/1
  Gain8/1 -> Bias1/1
  Bias/1 -> Gain8/1
  q/1 -> Bias/1

== system rlQuadrupedRobot/Observation/Subsystem8 ==
  f : Inport
  Gain8 : Gain  Gain=1/friction_force_max
  Sqrt : Sqrt
  Square : Math  Operator=square  SignedPower=on
  Sum of Elements : Sum  Inputs=+
  fhat : Outport  VectorParamsAs1DForOutWhenUnconnected=off
  wires:
  f/1 -> Gain8/1
  Gain8/1 -> Square/1
  Square/1 -> Sum of Elements/1
  Sum of Elements/1 -> Sqrt/1
  Sqrt/1 -> fhat/1

== system rlQuadrupedRobot/Observation/Subsystem9 ==
  f : Inport
  Gain8 : Gain  Gain=1/friction_force_max
  Sqrt : Sqrt
  Square : Math  Operator=square  SignedPower=on
  Sum of Elements : Sum  Inputs=+
  fhat : Outport  VectorParamsAs1DForOutWhenUnconnected=off
  wires:
  f/1 -> Gain8/1
  Gain8/1 -> Square/1
  Square/1 -> Sum of Elements/1
  Sum of Elements/1 -> Sqrt/1
  Sqrt/1 -> fhat/1
